simulink model "DTSMC"  (R2025a)
settings: Solver=VariableStepAuto  StartTime=0.0  StopTime=40  RelTol=1e-3
values from neighbouring files (symbols this model uses):
  p01 = [0 3.2 2]'    [paramDTSMC.m]
  p02 = [-1.6 0 2]'    [paramDTSMC.m]
  p03 = [1.6 0 2]'    [paramDTSMC.m]
settings Model: Creator=vinh1  LastModifiedBy=vinh1

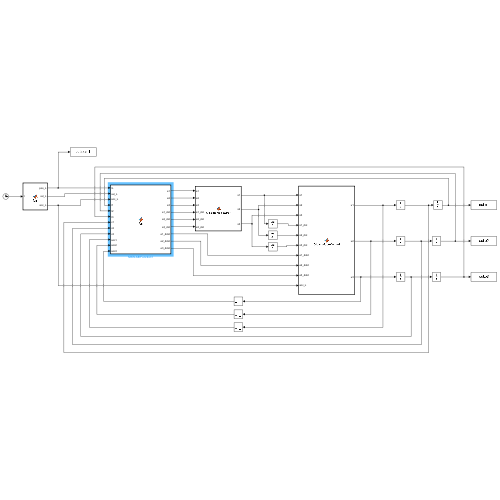
[thumbnail: Simulink's stored preview of the top-level diagram]
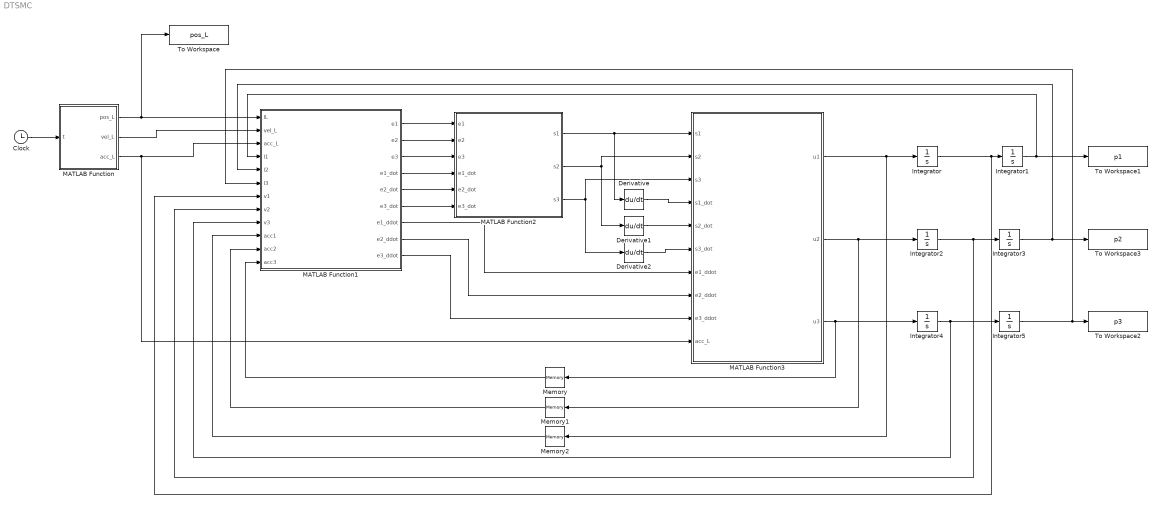
== system DTSMC ==
  Clock : Clock
      settings: Decimation=45
  Derivative : Derivative
  Derivative1 : Derivative
  Derivative2 : Derivative
  Integrator : Integrator  InitialCondition=zeros(3,1)
  Integrator1 : Integrator  InitialCondition=p01
  Integrator2 : Integrator  InitialCondition=zeros(3,1)
  Integrator3 : Integrator  InitialCondition=p02
  Integrator4 : Integrator  InitialCondition=zeros(3,1)
  Integrator5 : Integrator  InitialCondition=p03
  MATLAB Function : MATLAB Function  TreatAsAtomicUnit=on
  MATLAB Function1 : MATLAB Function  TreatAsAtomicUnit=on
  MATLAB Function2 : MATLAB Function  TreatAsAtomicUnit=on
  MATLAB Function3 : MATLAB Function  TreatAsAtomicUnit=on
  Memory : Memory
  Memory1 : Memory
  Memory2 : Memory
  To Workspace : ToWorkspace  VariableName=pos_L  SampleTime=-1
  To Workspace1 : ToWorkspace  VariableName=p1  SampleTime=-1
  To Workspace2 : ToWorkspace  VariableName=p3  SampleTime=-1
  To Workspace3 : ToWorkspace  VariableName=p2  SampleTime=-1
  wires:
  Clock/1 -> MATLAB Function/1(t)
  MATLAB Function1/1(e1) -> MATLAB Function2/1(e1)
  MATLAB Function1/2(e2) -> MATLAB Function2/2(e2)
  MATLAB Function1/3(e3) -> MATLAB Function2/3(e3)
  MATLAB Function/1(pos_L) -> MATLAB Function1/1(lL), To Workspace/1
  MATLAB Function/2(vel_L) -> MATLAB Function1/2(vel_L)
  MATLAB Function/3(acc_L) -> MATLAB Function1/3(acc_L), MATLAB Function3/10(acc_L)
  MATLAB Function3/1(u1) -> Memory2/1, Integrator/1
  Integrator/1 -> MATLAB Function1/7(v1), Integrator1/1
  Integrator4/1 -> MATLAB Function1/9(v3), Integrator5/1
  Integrator2/1 -> MATLAB Function1/8(v2), Integrator3/1
  Integrator1/1 -> MATLAB Function1/4(l1), To Workspace1/1
  Integrator3/1 -> MATLAB Function1/5(l2), To Workspace3/1
  Integrator5/1 -> MATLAB Function1/6(l3), To Workspace2/1
  MATLAB Function1/4(e1_dot) -> MATLAB Function2/4(e1_dot)
  MATLAB Function1/5(e2_dot) -> MATLAB Function2/5(e2_dot)
  MATLAB Function1/6(e3_dot) -> MATLAB Function2/6(e3_dot)
  MATLAB Function1/7(e1_ddot) -> MATLAB Function3/7(e1_ddot)
  MATLAB Function1/8(e2_ddot) -> MATLAB Function3/8(e2_ddot)
  MATLAB Function1/9(e3_ddot) -> MATLAB Function3/9(e3_ddot)
  MATLAB Function2/1(s1) -> MATLAB Function3/1(s1), Derivative/1
  MATLAB Function2/2(s2) -> Derivative1/1, MATLAB Function3/2(s2)
  MATLAB Function2/3(s3) -> MATLAB Function3/3(s3), Derivative2/1
  Derivative/1 -> MATLAB Function3/4(s1_dot)
  Derivative1/1 -> MATLAB Function3/5(s2_dot)
  Derivative2/1 -> MATLAB Function3/6(s3_dot)
  MATLAB Function3/3(u3) -> Memory/1, Integrator4/1
  Memory/1 -> MATLAB Function1/12(acc3)
  MATLAB Function3/2(u2) -> Memory1/1, Integrator2/1
  Memory1/1 -> MATLAB Function1/11(acc2)
  Memory2/1 -> MATLAB Function1/10(acc1)

== matlab function DTSMC/MATLAB Function1 ==
  data: lL input; vel_L input; acc_L input; l1 input; e1 output; e2 output; l2 input; l3 input; v1 input; v2 input; e3 output; v3 input; acc1 input; acc2 input; acc3 input; e1_dot output; e2_dot output; e3_dot output; e1_ddot output; e2_ddot output; e3_ddot output
function [e1, e2, e3, e1_dot, e2_dot, e3_dot, e1_ddot, e2_ddot, e3_ddot] = fcn(lL, vel_L, acc_L, l1, l2, l3, v1, v2, v3, acc1, acc2, acc3)

w = 2;

E1L = [0 5 -1]';
E2L = [-5 -5 -2]';

E12 = [5 10 1]';
E21 = [-5 -10 -1]';
E31 = [5 -10 -2]';
E32 = [10 0 -1]';

e1 = l1 - (1/w)*((lL + E1L) + (l2 + E12));
e2 = l2 - (1/w)*((lL + E2L) + (l1 + E21));
e3 = l3 - (1/w)*((l1 + E31) + (l2 + E32));

e1_dot = v1 - (1/w)*(vel_L + v2);
e2_dot = v2 - (1/w)*(vel_L + v1);
e3_dot = v3 - (1/w)*(v1 + v2);

e1_ddot = acc1 - (1/w)*(acc_L + acc2);
e2_ddot = acc2 - (1/w)*(acc_L + acc1);
e3_ddot = acc3 - (1/w)*(acc1 + acc2);

== matlab function DTSMC/MATLAB Function ==
  data: t input; pos_L output; vel_L output; acc_L output
function [pos_L, vel_L, acc_L]  = fcn(t)

x = 2*cos(t + pi/3);
y = 2*sin(t + pi/3);
z = 0.5*t +3;

pos_L = [x y z]';

x_dot = -2*sin(t + pi/3);
y_dot = 2*cos(t + pi/3);
z_dot = 0.5;

vel_L = [x_dot y_dot z_dot]';

x_ddot = -2*cos(t + pi/3);
y_ddot = -2*sin(t + pi/3);
z_ddot = 0;

acc_L = [x_ddot y_ddot z_ddot]';

== matlab function DTSMC/MATLAB Function2 ==
  data: e1 input; e2 input; e3 input; e1_dot input; s1 output; s2 output; e2_dot input; e3_dot input; s3 output
function [s1, s2, s3] = SlindingModeError(e1, e2, e3, e1_dot, e2_dot, e3_dot)

s1 = e1_dot + 3*sign(e1).*sqrt(abs(e1));
s2 = e2_dot + 3*sign(e2).*sqrt(abs(e2));
s3 = e3_dot + 3*sign(e3).*sqrt(abs(e3));

== matlab function DTSMC/MATLAB Function3 ==
  data: s1 input; s2 input; s3 input; s1_dot input; s2_dot input; s3_dot input; e1_ddot input; e2_ddot input; e3_ddot input; acc_L input; u1 output size=[3,1]; u2 output size=[3,1]; u3 output size=[3,1]
function [u1, u2, u3] = SlidingModeControl(s1, s2, s3, s1_dot, s2_dot, s3_dot, e1_ddot, e2_ddot, e3_ddot, acc_L)

omegai = 2;
Hi = diag([3 3 3]);
Ki = diag([2 2 2]);


w1 = (s1_dot - e1_ddot)*2/3;
w2 = (s2_dot - e2_ddot)*2/3;
w3 = (s3_dot - e3_ddot)*2/3;

u1 = (1/omegai)*acc_L - (1/2)*3*w1 - 2*sign(s1);
u2 = (1/omegai)*acc_L - (1/2)*3*w2 - 2*sign(s2);
u3 = -(1/2)*3*w3 - 2*sign(s3);
